simulink model "assignment5"  (R2026a)
settings: Solver=VariableStepAuto  StopTime=7.5  MaxStep=0.01
values from neighbouring files (symbols this model uses):
  E1 = 2    [assignment5_param.m]
  E2 = 1    [assignment5_param.m]
  omega1 = 0.5    [assignment5_param.m]
  omega2 = 2    [assignment5_param.m]
settings Model: Creator=saradenti  LastModifiedBy=saradenti

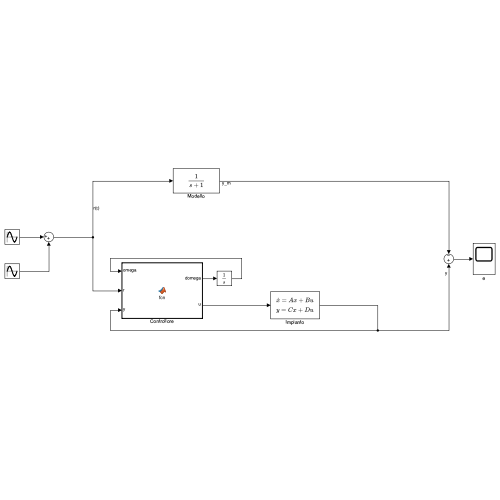
[thumbnail: Simulink's stored preview of the top-level diagram]
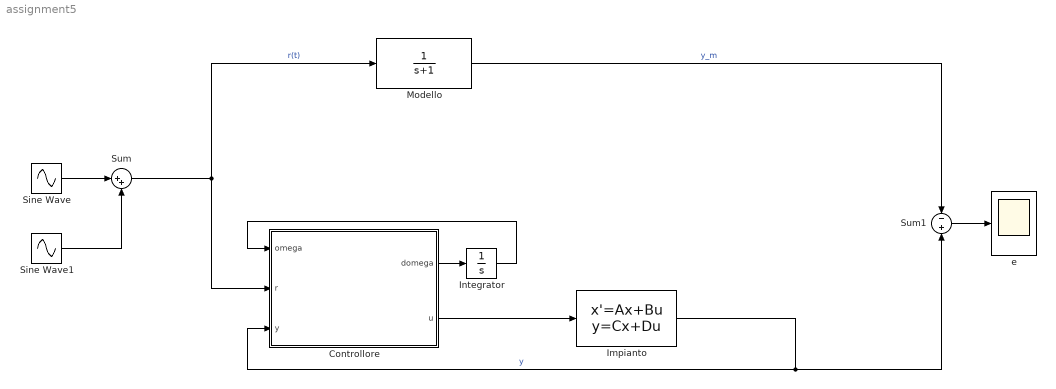
== system assignment5 ==
  Controllore : MATLAB Function  TreatAsAtomicUnit=on
  Impianto : StateSpace  A=[10 -5; 1 0]  B=[1; 0]  C=[1 2]  D=0  InitialCondition=[10; 10]
  Integrator : Integrator
  Modello : TransferFcn  Denominator=[1 1]
  Sine Wave : Sin  Amplitude=E1  Frequency=omega1  SampleTime=0
  Sine Wave1 : Sin  Amplitude=E2  Frequency=omega2  SampleTime=0
  Sum : Sum  Inputs=|++
  Sum1 : Sum  Inputs=-|+
  e : Scope
      settings: ActiveDisplayYMinimum=-69.309800744590888  ActiveDisplayYMaximum=41.034422304954539
  wires:
  Sine Wave/1 -> Sum/1
  Sine Wave1/1 -> Sum/2
  Sum/1 -> Controllore/2(r), Modello/1  "r(t)"
  Modello/1 -> Sum1/1  "y_m"
  Controllore/1(domega) -> Integrator/1
  Integrator/1 -> Controllore/1(omega)
  Impianto/1 -> Sum1/2, Controllore/3(y)  "y"
  Sum1/1 -> e/1
  Controllore/2(u) -> Impianto/1

== matlab function assignment5/Controllore ==
  data: domega output; omega input; r input; y input; u output
function [domega, u] = fcn(omega, r, y)

    u = 29 * omega - 13 * y + r;
    domega = - 2 * omega + y;
